simulink model "pgfm_ctrl_analysis"  (R2026b)
settings: Solver=ode23t  StopTime=param.sim.simlength  FixedStep=param.sim.tc  MaxStep=param.glb_time.tc  RelTol=1e-4
values from neighbouring files (symbols this model uses):
  param = add_template_extras(param, options)    [init_model.m]
undefined symbols (not defined in the file or in its folder): magnitude
libraries: fl_lib x99, nesl_utility x59, afe_uvw_ctrl x15, discrete_time_low_pass_filter x3, threephase_inductor_lib x3, dclink_for_two_levels x3, three_phase_pwm_modulator x3, ideal_bridges_lib x3, lithium_ion_battery x1, three_phase_voltage_with_frt_emulator_mfcn x1
(part 1 of 6)
settings Model: Creator=dbagn  LastModifiedBy=dbagn
settings SolverCC: SolverResetMethod=Robust  ZeroCrossControl=DisableAll
settings DataIOCC: DSMLogging=off  ReturnWorkspaceOutputs=off  SaveOutput=off  SaveTime=off  SignalLogging=off
settings OptimizationCC: ReuseModelBlockBuffer=off
settings SFSimCC: CustomCodeUndefinedFunction=ThrowError  DefaultCustomCodeDeterministicFunctions=All
settings SFSimCC: SimCustomHeaderCode=|
  | #include "rpi.h"
  | #include "rpi_simulink.h"
  | #include "bemf_obsv_load_est.h"
  | #include "bemf_obsv_load_est_simulink.h"
  | #include "dqpll_grid.h"
  | #include "dsmavgflt.h"
  | #include "bemf_obsv.h"
  | #include "bemf_obsv_simulink.h"
  | #include "mavgflt.h"
  | #include "mavgflt_simulink.h"
  | #include "mavgflts.h"
  | #include "mavgflts_simulink.h"
  | #include "sv_pwm_cm.h"
  | #include "dsmavgflt_simulink.h"
  | #include "linear_double_integrator_observer_simulink.h"
  | #include "sv_pwm_cm_simulink.h"
  | #include "dqvector_pi.h"
  | #include "dqpll_grid_simulink.h"
  | #include "first_harmonic_tracker.h"
  | #include "dqvector_pi_simulink.h"
  | #include "first_harmonic_tracker_simulink.h"
  | #include "dqpll_thyr.h"
  | #include "sv_pwm_simulink.h"
  | #include "sv_pwm.h"
  | #include "dqpll_thyr_simulink.h"
  | #include "linear_double_integrator_observer.h"
  | #include "math_f.h"
settings SFSimCC: SimUserIncludeDirs=|
  | include
  | src
settings SFSimCC: SimUserSources=|
  | "rpi.c"
  | "rpi_simulink.c"
  | "mavgflt_simulink.c"
  | "mavgflt.c"
  | "mavgflts_simulink.c"
  | "mavgflts.c"
  | "dsmavgflt_simulink.c"
  | "dsmavgflt.c"
  | "bemf_obsv_simulink.c"
  | "bemf_obsv.c"
  | "bemf_obsv_load_est_simulink.c"
  | "bemf_obsv_load_est.c"
  | "dqvector_pi.c"
  | "dqvector_pi_simulink.c"
  | "sv_pwm_simulink.c"
  | "sv_pwm.c"
  | "first_harmonic_tracker_simulink.c"
  | "first_harmonic_tracker.c"
  | "dqpll_thyr_simulink.c"
  | "dqpll_thyr.c"
  | "dqpll_grid_simulink.c"
  | "dqpll_grid.c"
  | "linear_double_integrator_observer_simulink.c"
  | "linear_double_integrator_observer.c"
  | "sv_pwm_cm_simulink.c"
  | "sv_pwm_cm.c"
settings RTWCC: DLArmComputeVersion=19.05
settings SimscapeCC: SimscapeUseEnergyAccounting=off

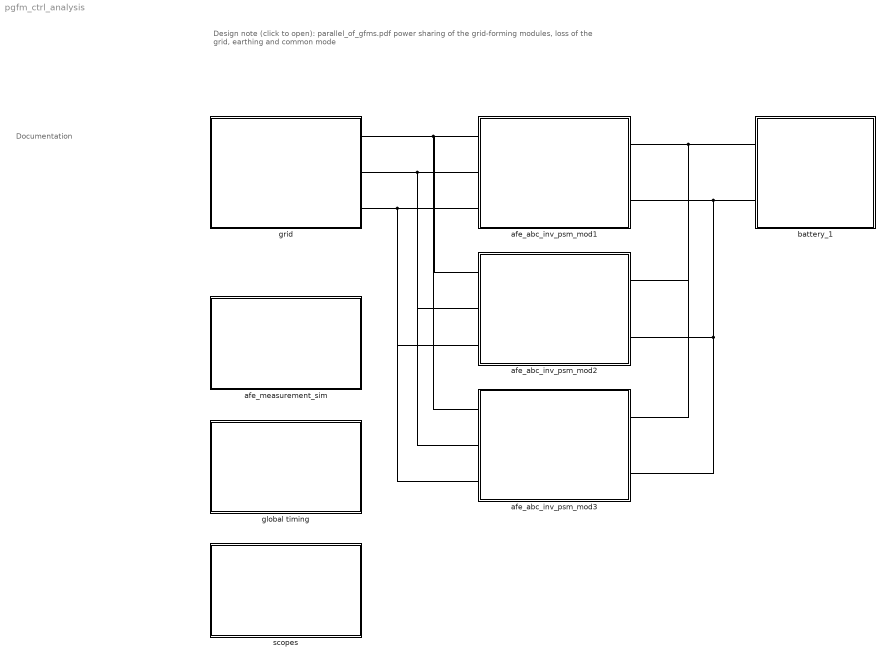
== system pgfm_ctrl_analysis ==
  note: Documentation
  note: Design note (click to open): parallel_of_gfms.pdf
      | power sharing of the grid-forming modules, loss of the grid, earthing and common mode
  afe_abc_inv_psm_mod1 : Subsystem
  afe_abc_inv_psm_mod2 : Subsystem
  afe_abc_inv_psm_mod3 : Subsystem
  afe_measurement_sim : Subsystem
  battery_1 : Subsystem
  global timing : Subsystem
  grid : Subsystem
  scopes : Subsystem
  connections:
  grid/RConn1 -- afe_abc_inv_psm_mod3/LConn1 -- afe_abc_inv_psm_mod2/LConn1 -- afe_abc_inv_psm_mod1/LConn1
  grid/RConn3 -- afe_abc_inv_psm_mod3/LConn3 -- afe_abc_inv_psm_mod2/LConn3 -- afe_abc_inv_psm_mod1/LConn3
  afe_abc_inv_psm_mod1/LConn2 -- afe_abc_inv_psm_mod3/LConn2 -- afe_abc_inv_psm_mod2/LConn2 -- grid/RConn2
  battery_1/RConn1 -- afe_abc_inv_psm_mod3/RConn1 -- afe_abc_inv_psm_mod2/RConn1 -- afe_abc_inv_psm_mod1/RConn1
  battery_1/RConn2 -- afe_abc_inv_psm_mod3/RConn2 -- afe_abc_inv_psm_mod2/RConn2 -- afe_abc_inv_psm_mod1/RConn2

== system pgfm_ctrl_analysis/afe_abc_inv_psm_mod1 ==
  AFE_control : Subsystem
  LCL_filter : Subsystem
  afe : Subsystem
  ug_a : PMIOPort  Side=Left
  ug_b : PMIOPort  Port=2  Side=Left
  ug_c : PMIOPort  Port=3  Side=Left
  Udc(+) : PMIOPort  Port=4  Side=Right
  Udc(-) : PMIOPort  Port=5  Side=Right
  wires:
  AFE_control/1(dabc_out) -> afe/1(dabc)
  connections:
  LCL_filter/LConn1 -- afe/LConn1
  LCL_filter/LConn2 -- afe/LConn2
  LCL_filter/LConn3 -- afe/LConn3
  ug_a/RConn1 -- LCL_filter/RConn1
  ug_b/RConn1 -- LCL_filter/RConn2
  ug_c/RConn1 -- LCL_filter/RConn3
  Udc(+)/RConn1 -- afe/RConn1
  afe/RConn2 -- Udc(-)/RConn1

== system pgfm_ctrl_analysis/afe_abc_inv_psm_mod2 ==
  AFE_control : Subsystem
  LCL_filter : Subsystem
  afe : Subsystem
  ug_a : PMIOPort  Side=Left
  ug_b : PMIOPort  Port=2  Side=Left
  ug_c : PMIOPort  Port=3  Side=Left
  Udc(+) : PMIOPort  Port=4  Side=Right
  Udc(-) : PMIOPort  Port=5  Side=Right
  wires:
  AFE_control/1(dabc_out) -> afe/1(dabc)
  connections:
  afe/RConn2 -- Udc(-)/RConn1
  Udc(+)/RConn1 -- afe/RConn1
  ug_c/RConn1 -- LCL_filter/RConn3
  ug_b/RConn1 -- LCL_filter/RConn2
  ug_a/RConn1 -- LCL_filter/RConn1
  LCL_filter/LConn3 -- afe/LConn3
  LCL_filter/LConn2 -- afe/LConn2
  LCL_filter/LConn1 -- afe/LConn1

== system pgfm_ctrl_analysis/afe_abc_inv_psm_mod3 ==
  AFE_control : Subsystem
  LCL_filter : Subsystem
  afe : Subsystem
  ug_a : PMIOPort  Side=Left
  ug_b : PMIOPort  Port=2  Side=Left
  ug_c : PMIOPort  Port=3  Side=Left
  Udc(+) : PMIOPort  Port=4  Side=Right
  Udc(-) : PMIOPort  Port=5  Side=Right
  wires:
  AFE_control/1(dabc_out) -> afe/1(dabc)
  connections:
  LCL_filter/LConn1 -- afe/LConn1
  LCL_filter/LConn2 -- afe/LConn2
  LCL_filter/LConn3 -- afe/LConn3
  ug_a/RConn1 -- LCL_filter/RConn1
  ug_b/RConn1 -- LCL_filter/RConn2
  ug_c/RConn1 -- LCL_filter/RConn3
  Udc(+)/RConn1 -- afe/RConn1
  afe/RConn2 -- Udc(-)/RConn1

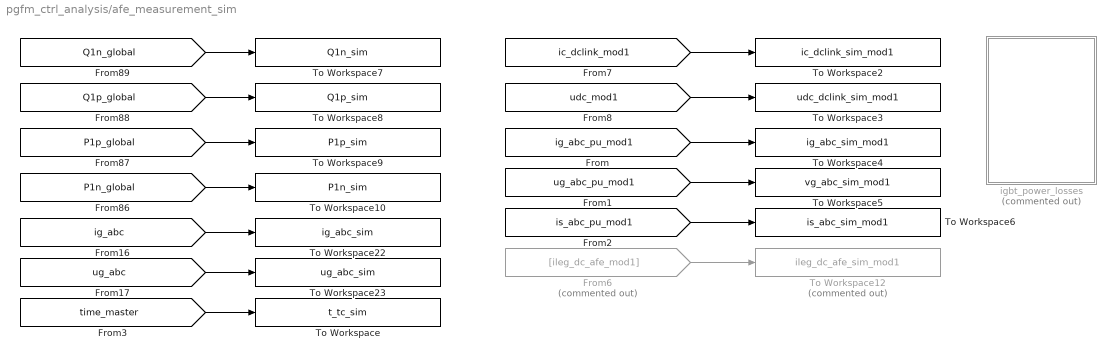
== system pgfm_ctrl_analysis/afe_measurement_sim ==
  From6 : From  Commented=on  GotoTag=ileg_dc_afe_mod1
  To Workspace : ToWorkspace  VariableName=t_tc_sim  SampleTime=param.glb_time.tc
      settings: MaxDataPoints=param.glb_time.Nc
  To Workspace10 : ToWorkspace  VariableName=P1n_sim  SampleTime=param.glb_time.ts_afe
      settings: MaxDataPoints=param.glb_time.Ns_afe
  To Workspace12 : ToWorkspace  Commented=on  VariableName=ileg_dc_afe_sim_mod1  SampleTime=param.glb_time.tc
      settings: MaxDataPoints=param.glb_time.Nc
  To Workspace2 : ToWorkspace  VariableName=ic_dclink_sim_mod1  SampleTime=param.glb_time.tc
      settings: MaxDataPoints=param.glb_time.Nc
  To Workspace22 : ToWorkspace  VariableName=ig_abc_sim  SampleTime=param.glb_time.tc
      settings: MaxDataPoints=param.glb_time.Nc
  To Workspace23 : ToWorkspace  VariableName=ug_abc_sim  SampleTime=param.glb_time.tc
      settings: MaxDataPoints=param.glb_time.Nc
  To Workspace3 : ToWorkspace  VariableName=udc_dclink_sim_mod1  SampleTime=param.glb_time.tc
      settings: MaxDataPoints=param.glb_time.Nc
  To Workspace4 : ToWorkspace  VariableName=ig_abc_sim_mod1  SampleTime=param.glb_time.tc
      settings: MaxDataPoints=param.glb_time.Nc
  To Workspace5 : ToWorkspace  VariableName=vg_abc_sim_mod1  SampleTime=param.glb_time.tc
      settings: MaxDataPoints=param.glb_time.Nc
  To Workspace6 : ToWorkspace  VariableName=is_abc_sim_mod1  SampleTime=param.glb_time.tc
      settings: MaxDataPoints=param.glb_time.Nc
  To Workspace7 : ToWorkspace  VariableName=Q1n_sim  SampleTime=param.glb_time.ts_afe
      settings: MaxDataPoints=param.glb_time.Ns_afe
  To Workspace8 : ToWorkspace  VariableName=Q1p_sim  SampleTime=param.glb_time.ts_afe
      settings: MaxDataPoints=param.glb_time.Ns_afe
  To Workspace9 : ToWorkspace  VariableName=P1p_sim  SampleTime=param.glb_time.ts_afe
      settings: MaxDataPoints=param.glb_time.Ns_afe
  igbt_power_losses : Subsystem  Commented=on
  wires:
  [time_master] -> To Workspace/1
  [Q1n_global] -> To Workspace7/1
  [Q1p_global] -> To Workspace8/1
  [P1p_global] -> To Workspace9/1
  [P1n_global] -> To Workspace10/1
  [ug_abc] -> To Workspace23/1
  [ig_abc] -> To Workspace22/1
  [ug_abc_pu_mod1] -> To Workspace5/1
  [ig_abc_pu_mod1] -> To Workspace4/1
  From6/1 -> To Workspace12/1
  [udc_mod1] -> To Workspace3/1
  [ic_dclink_mod1] -> To Workspace2/1
  [is_abc_pu_mod1] -> To Workspace6/1

== system pgfm_ctrl_analysis/battery_1 ==
  Electrical Reference1 : fl_lib/Electrical/Electrical Elements/Electrical Reference
  HF and Ground Network : Subsystem
  To Workspace14 : ToWorkspace  VariableName=battery_1_data_sim  SampleTime=param.glb_time.tc
      settings: MaxDataPoints=param.glb_time.Nc  Decimation=param.glb_time.decimation_tc
  lithium ion battery : Scope
      settings: ActiveDisplayYMinimum=-3613.5737689566768  ActiveDisplayYMaximum=22003.145712945909  DataLoggingVariableName=ScopeData3
  lithium_ion_battery : lithium_ion_battery/lithium_ion_battery  Q=param.battery.pack_1.Q  number_of_cells=param.battery.pack_1.number_of_cells  E_1=param.battery.pack_1.E_1  E0=param.battery.pack_1.E0  E1=param.battery.pack_1.E1  E2=param.battery.pack_1.E2  E3=param.battery.pack_1.E3  Elog=param.battery.pack_1.Elog  R0=param.battery.pack_1.R0  R1=param.battery.pack_1.R1  C1=param.battery.pack_1.C1  M=param.battery.pack_1.M  alpha=param.battery.pack_1.alpha  soc_init=param.battery.pack_1.soc_init  ts_battery=param.glb_time.ts_dab  q1Kalman=param.battery.pack_1.q1Kalman  q2Kalman=param.battery.pack_1.q2Kalman  q3Kalman=param.battery.pack_1.q3Kalman  rKalman=param.battery.pack_1.rKalman  tc=param.glb_time.tc  enable_white_noise_m=0  battery_voltage_init_m=param.battery.nominal_battery_voltage_1
  single_phase_ui_measure : Subsystem
  dc(+) : PMIOPort  Side=Right
  dc(-) : PMIOPort  Port=2  Side=Right
  wires:
  lithium_ion_battery/1 -> To Workspace14/1, lithium ion battery/1
  connections:
  single_phase_ui_measure/RConn1 -- dc(+)/RConn1
  single_phase_ui_measure/LConn1 -- HF and Ground Network/LConn1 -- lithium_ion_battery/RConn1
  dc(-)/RConn1 -- single_phase_ui_measure/RConn2
  single_phase_ui_measure/LConn2 -- HF and Ground Network/LConn2 -- lithium_ion_battery/RConn2
  HF and Ground Network/RConn1 -- Electrical Reference1/LConn1

== system pgfm_ctrl_analysis/global timing ==
  Unit Delay : UnitDelay  SampleTime=param.glb_time.tc
  Unit Delay1 : UnitDelay  SampleTime=param.glb_time.tc
  Unit Delay2 : UnitDelay  SampleTime=param.glb_time.tc
  time_afe1 : Subsystem  mask{k=param.afe.behav.time_gain_module_1}
      mask prompts: k "Time Gain"
      mask Display:
      | disp('time-gen');
      | port_label('input', 1, 'crt');
      | port_label('output', 1, 'tout');
  time_afe2 : Subsystem  mask{k=param.afe.behav.time_gain_module_2}
      mask prompts: k "Time Gain"
      mask Display:
      | disp('time-gen');
      | port_label('input', 1, 'crt');
      | port_label('output', 1, 'tout');
  time_afe3 : Subsystem  mask{k=param.afe.behav.time_gain_module_3}
      mask prompts: k "Time Gain"
      mask Display:
      | disp('time-gen');
      | port_label('input', 1, 'crt');
      | port_label('output', 1, 'tout');
  time_master : Subsystem  mask{k=1}
      mask prompts: k "Time Gain"
      mask Display:
      | disp('time-gen');
      | port_label('output', 1, 'tout');
  tag scope: time_afe_module_1=global, time_afe_module_2=global, time_afe_module_3=global, time_master=global
  wires:
  time_afe1/1(Out1) -> [time_afe_module_1]
  time_afe2/1(Out1) -> [time_afe_module_2]
  time_master/1(Out1) -> [time_master]
  [local_time_corr_afe1] -> Unit Delay/1
  Unit Delay/1 -> time_afe1/1(correction_time)
  [local_time_corr_afe2] -> Unit Delay1/1
  Unit Delay1/1 -> time_afe2/1(correction_time)
  [local_time_corr_afe3] -> Unit Delay2/1
  Unit Delay2/1 -> time_afe3/1(correction_time)
  time_afe3/1(Out1) -> [time_afe_module_3]

== system pgfm_ctrl_analysis/grid ==
  grid_emulator : Subsystem
  power meter iec mfunc : Subsystem
  threephase_vi_measures : Subsystem
  ua : PMIOPort  Side=Right
  ub : PMIOPort  Port=2  Side=Right
  uc : PMIOPort  Port=3  Side=Right
  connections:
  threephase_vi_measures/LConn3 -- grid_emulator/RConn3
  threephase_vi_measures/LConn1 -- grid_emulator/RConn1
  threephase_vi_measures/RConn2 -- ub/RConn1
  threephase_vi_measures/LConn2 -- grid_emulator/RConn2
  threephase_vi_measures/RConn1 -- ua/RConn1
  threephase_vi_measures/RConn3 -- uc/RConn1

== system pgfm_ctrl_analysis/scopes ==
  grid_afe_side : Subsystem
  igbt_power_losses : Subsystem  Commented=on
  mosfet_power_losses : Subsystem  Commented=on

== system pgfm_ctrl_analysis/afe_abc_inv_psm_mod1/AFE_control ==
  To Workspace : ToWorkspace  VariableName=afe_ctrl_data_output_mod1  SampleTime=param.glb_time.ts_afe
      settings: MaxDataPoints=param.glb_time.Ns_afe
  afe_control : Subsystem
  dabc_out : Outport
  tag scope: local_time_corr_afe1=global
  wires:
  [TRGO_afe_module_1] -> afe_control/Trigger
  [ug_abc_pu_mod1] -> afe_control/1(ug_abc_pu)
  [is_abc_pu_mod1] -> afe_control/4(is_abc_pu)
  [vdc_pu_afe_mod1] -> afe_control/2(udc_pu)
  afe_control/1(duvw) -> dabc_out/1
  [ig_abc_pu_mod1] -> afe_control/3(ig_abc_pu)
  [time_afe_module_1] -> afe_control/5(local_time)
  [time_master] -> afe_control/6(master_time)
  [phase_grid_emulator] -> afe_control/7(grid_phase)
  afe_control/3(m_data) -> To Workspace/1
  afe_control/2(AFE1_local_time_corr) -> [local_time_corr_afe1]

== system pgfm_ctrl_analysis/afe_abc_inv_psm_mod1/LCL_filter ==
  CFu1 : fl_lib/Electrical/Electrical Elements/Capacitor  c=param.afe.hw.CFu F  r=param.afe.hw.RCFu Ohm  g=0 1/Ohm  i_specify=off  i_priority=None  i=0 A  i_nominal_specify=off  i_nominal_value=1  i_nominal_unit=A  v_specify=off  v_priority=None  v=0 V  v_nominal_specify=off  v_nominal_value=1  v_nominal_unit=V  vc_specify=off  vc_priority=High  vc=0 V  vc_nominal_specify=off  vc_nominal_value=1  vc_nominal_unit=V
  CFu2 : fl_lib/Electrical/Electrical Elements/Capacitor  c=param.afe.hw.CFu F  r=param.afe.hw.RCFu Ohm  g=0 1/Ohm  i_specify=off  i_priority=None  i=0 A  i_nominal_specify=off  i_nominal_value=1  i_nominal_unit=A  v_specify=off  v_priority=None  v=0 V  v_nominal_specify=off  v_nominal_value=1  v_nominal_unit=V  vc_specify=off  vc_priority=High  vc=0 V  vc_nominal_specify=off  vc_nominal_value=1  vc_nominal_unit=V
  CFu3 : fl_lib/Electrical/Electrical Elements/Capacitor  c=param.afe.hw.CFu F  r=param.afe.hw.RCFu Ohm  g=0 1/Ohm  i_specify=off  i_priority=None  i=0 A  i_nominal_specify=off  i_nominal_value=1  i_nominal_unit=A  v_specify=off  v_priority=None  v=0 V  v_nominal_specify=off  v_nominal_value=1  v_nominal_unit=V  vc_specify=off  vc_priority=High  vc=0 V  vc_nominal_specify=off  vc_nominal_value=1  vc_nominal_unit=V
  Inductor : fl_lib/Electrical/Electrical Elements/Inductor  l=1e-6 H  r=0 Ohm  g=1e-9 1/Ohm  i_specify=on  i_priority=High  i=0 A  i_nominal_specify=off  i_nominal_value=1  i_nominal_unit=A  v_specify=off  v_priority=None  v=0 V  v_nominal_specify=off  v_nominal_value=1  v_nominal_unit=V  i_L_specify=off  i_L_priority=High  i_L=0 A  i_L_nominal_specify=off  i_L_nominal_value=1  i_L_nominal_unit=A
  Inductor1 : fl_lib/Electrical/Electrical Elements/Inductor  l=1e-6 H  r=0 Ohm  g=1e-9 1/Ohm  i_specify=on  i_priority=High  i=0 A  i_nominal_specify=off  i_nominal_value=1  i_nominal_unit=A  v_specify=off  v_priority=None  v=0 V  v_nominal_specify=off  v_nominal_value=1  v_nominal_unit=V  i_L_specify=off  i_L_priority=High  i_L=0 A  i_L_nominal_specify=off  i_L_nominal_value=1  i_L_nominal_unit=A
  Inductor2 : fl_lib/Electrical/Electrical Elements/Inductor  l=1e-6 H  r=0 Ohm  g=1e-9 1/Ohm  i_specify=on  i_priority=High  i=0 A  i_nominal_specify=off  i_nominal_value=1  i_nominal_unit=A  v_specify=off  v_priority=None  v=0 V  v_nominal_specify=off  v_nominal_value=1  v_nominal_unit=V  i_L_specify=off  i_L_priority=High  i_L=0 A  i_L_nominal_specify=off  i_L_nominal_value=1  i_L_nominal_unit=A
  threephase inductor : threephase_inductor_lib/threephase inductor  Lp=param.afe.hw.LFu H  L0=param.afe.hw.LFu_cm H  Rp=param.afe.hw.RLFu Ohm  R0=param.afe.hw.RLFu_cm Ohm  Lls=5e-6 H  uu_1_specify=off  uu_1_priority=None  uu_1=0 V  uu_1_nominal_specify=off  uu_1_nominal_value=1  uu_1_nominal_unit=V  uv_1_specify=off  uv_1_priority=None  uv_1=0 V  uv_1_nominal_specify=off  uv_1_nominal_value=1  uv_1_nominal_unit=V  uw_1_specify=off  uw_1_priority=None  uw_1=0 V  uw_1_nominal_specify=off  uw_1_nominal_value=1  uw_1_nominal_unit=V  uu_2_specify=off  uu_2_priority=None  uu_2=0 V  uu_2_nominal_specify=off  uu_2_nominal_value=1  uu_2_nominal_unit=V  uv_2_specify=off  uv_2_priority=None  uv_2=0 V  uv_2_nominal_specify=off  uv_2_nominal_value=1  uv_2_nominal_unit=V  uw_2_specify=off  uw_2_priority=None  uw_2=0 V  uw_2_nominal_specify=off  uw_2_nominal_value=1  uw_2_nominal_unit=V  iu_specify=off  iu_priority=High  iu=0 A  iu_nominal_specify=off  iu_nominal_value=1  iu_nominal_unit=A  iv_specify=off  iv_priority=High  iv=0 A  iv_nominal_specify=off  iv_nominal_value=1  iv_nominal_unit=A  iw_specify=off  iw_priority=High  iw=0 A  iw_nominal_specify=off  iw_nominal_value=1  iw_nominal_unit=A
  threephase_vi_measures_stack : Subsystem
  threephase_vi_measures_stack1 : Subsystem
  us_a : PMIOPort  Side=Left
  ug_a : PMIOPort  Port=2  Side=Right
  us_b : PMIOPort  Port=3  Side=Left
  ug_b : PMIOPort  Port=4  Side=Right
  us_c : PMIOPort  Port=5  Side=Left
  ug_c : PMIOPort  Port=6  Side=Right
  connections:
  CFu1/RConn1 -- CFu3/RConn1 -- CFu2/RConn1
  Inductor/RConn1 -- threephase_vi_measures_stack1/LConn1 -- CFu1/LConn1
  Inductor2/RConn1 -- CFu3/LConn1 -- threephase_vi_measures_stack1/LConn3
  Inductor1/RConn1 -- CFu2/LConn1 -- threephase_vi_measures_stack1/LConn2
  threephase_vi_measures_stack/LConn1 -- us_a/RConn1
  threephase_vi_measures_stack/LConn2 -- us_b/RConn1
  threephase_vi_measures_stack/LConn3 -- us_c/RConn1
  threephase_vi_measures_stack/RConn1 -- threephase inductor/LConn1
  threephase_vi_measures_stack/RConn2 -- threephase inductor/LConn2
  threephase_vi_measures_stack/RConn3 -- threephase inductor/LConn3
  threephase inductor/RConn1 -- Inductor/LConn1
  Inductor1/LConn1 -- threephase inductor/RConn2
  Inductor2/LConn1 -- threephase inductor/RConn3
  ug_a/RConn1 -- threephase_vi_measures_stack1/RConn1
  ug_b/RConn1 -- threephase_vi_measures_stack1/RConn2
  ug_c/RConn1 -- threephase_vi_measures_stack1/RConn3

== system pgfm_ctrl_analysis/afe_abc_inv_psm_mod1/afe ==
  dabc : Inport
  Bus Selector : BusSelector  OutputSignals=vdc_pu
  Bus Selector1 : BusSelector  OutputSignals=udc,udc_p_gnd,udc_centertap_gnd,udc_n_gnd  OutputAsBus=on
  Bus Selector2 : BusSelector  OutputSignals=udc
  Bus Selector3 : BusSelector  OutputSignals=Cdc1_current
  dclink1 : dclink_for_two_levels/dclink  Cdc=param.afe.hw.CFi  Rudc_measure=1e6  Vdc_scale=param.afe.hw.udc_nom
  sv_pwm : Subsystem
  three_phase_inverter_ideal_switch_based_model : Subsystem
  us_a : PMIOPort  Side=Left
  us_b : PMIOPort  Port=2  Side=Left
  us_c : PMIOPort  Port=3  Side=Left
  Udc(+) : PMIOPort  Port=4  Side=Right
  Udc(-) : PMIOPort  Port=5  Side=Right
  tag scope: all_voltages_about_dclink=global, ic_dclink_mod1=global, udc_mod1=global, vdc_pu_afe_mod1=global, vdc_pu_inv_mod1=global
  wires:
  dabc/1 -> sv_pwm/1(duties_uvw)
  sv_pwm/1(gate_cmds) -> three_phase_inverter_ideal_switch_based_model/1(gate_commands)
  dclink1/1 -> Bus Selector1/1, Bus Selector2/1, Bus Selector3/1, Bus Selector/1
  Bus Selector1/1 -> [all_voltages_about_dclink]
  Bus Selector/1 -> [vdc_pu_afe_mod1], [vdc_pu_inv_mod1]  "<vdc_pu>"
  Bus Selector2/1 -> [udc_mod1]  "<udc>"
  Bus Selector3/1 -> [ic_dclink_mod1]  "<Cdc1_current>"
  connections:
  three_phase_inverter_ideal_switch_based_model/RConn2 -- us_b/RConn1
  dclink1/RConn1 -- Udc(+)/RConn1
  dclink1/RConn2 -- Udc(-)/RConn1
  three_phase_inverter_ideal_switch_based_model/RConn1 -- us_a/RConn1
  three_phase_inverter_ideal_switch_based_model/RConn3 -- us_c/RConn1
  dclink1/LConn2 -- three_phase_inverter_ideal_switch_based_model/LConn2
  dclink1/LConn1 -- three_phase_inverter_ideal_switch_based_model/LConn1

== system pgfm_ctrl_analysis/afe_abc_inv_psm_mod2/AFE_control ==
  To Workspace : ToWorkspace  VariableName=afe_ctrl_data_output_mod2  SampleTime=param.glb_time.ts_afe
      settings: MaxDataPoints=param.glb_time.Ns_afe
  afe_control : Subsystem
  dabc_out : Outport
  tag scope: local_time_corr_afe2=global
  wires:
  afe_control/2(AFE1_local_time_corr) -> [local_time_corr_afe2]
  afe_control/3(m_data) -> To Workspace/1
  [phase_grid_emulator] -> afe_control/7(grid_phase)
  [time_master] -> afe_control/6(master_time)
  [time_afe_module_2] -> afe_control/5(local_time)
  [ig_abc_pu_mod2] -> afe_control/3(ig_abc_pu)
  afe_control/1(duvw) -> dabc_out/1
  [vdc_pu_afe_mod2] -> afe_control/2(udc_pu)
  [is_abc_pu_mod2] -> afe_control/4(is_abc_pu)
  [ug_abc_pu_mod2] -> afe_control/1(ug_abc_pu)
  [TRGO_afe_module_2] -> afe_control/Trigger

== system pgfm_ctrl_analysis/afe_abc_inv_psm_mod2/LCL_filter ==
  CFu1 : fl_lib/Electrical/Electrical Elements/Capacitor  c=param.afe.hw.CFu F  r=param.afe.hw.RCFu Ohm  g=0 1/Ohm  i_specify=off  i_priority=None  i=0 A  i_nominal_specify=off  i_nominal_value=1  i_nominal_unit=A  v_specify=off  v_priority=None  v=0 V  v_nominal_specify=off  v_nominal_value=1  v_nominal_unit=V  vc_specify=off  vc_priority=High  vc=0 V  vc_nominal_specify=off  vc_nominal_value=1  vc_nominal_unit=V
  CFu2 : fl_lib/Electrical/Electrical Elements/Capacitor  c=param.afe.hw.CFu F  r=param.afe.hw.RCFu Ohm  g=0 1/Ohm  i_specify=off  i_priority=None  i=0 A  i_nominal_specify=off  i_nominal_value=1  i_nominal_unit=A  v_specify=off  v_priority=None  v=0 V  v_nominal_specify=off  v_nominal_value=1  v_nominal_unit=V  vc_specify=off  vc_priority=High  vc=0 V  vc_nominal_specify=off  vc_nominal_value=1  vc_nominal_unit=V
  CFu3 : fl_lib/Electrical/Electrical Elements/Capacitor  c=param.afe.hw.CFu F  r=param.afe.hw.RCFu Ohm  g=0 1/Ohm  i_specify=off  i_priority=None  i=0 A  i_nominal_specify=off  i_nominal_value=1  i_nominal_unit=A  v_specify=off  v_priority=None  v=0 V  v_nominal_specify=off  v_nominal_value=1  v_nominal_unit=V  vc_specify=off  vc_priority=High  vc=0 V  vc_nominal_specify=off  vc_nominal_value=1  vc_nominal_unit=V
  Inductor : fl_lib/Electrical/Electrical Elements/Inductor  l=1e-6 H  r=0 Ohm  g=1e-9 1/Ohm  i_specify=on  i_priority=High  i=0 A  i_nominal_specify=off  i_nominal_value=1  i_nominal_unit=A  v_specify=off  v_priority=None  v=0 V  v_nominal_specify=off  v_nominal_value=1  v_nominal_unit=V  i_L_specify=off  i_L_priority=High  i_L=0 A  i_L_nominal_specify=off  i_L_nominal_value=1  i_L_nominal_unit=A
  Inductor1 : fl_lib/Electrical/Electrical Elements/Inductor  l=1e-6 H  r=0 Ohm  g=1e-9 1/Ohm  i_specify=on  i_priority=High  i=0 A  i_nominal_specify=off  i_nominal_value=1  i_nominal_unit=A  v_specify=off  v_priority=None  v=0 V  v_nominal_specify=off  v_nominal_value=1  v_nominal_unit=V  i_L_specify=off  i_L_priority=High  i_L=0 A  i_L_nominal_specify=off  i_L_nominal_value=1  i_L_nominal_unit=A
  Inductor2 : fl_lib/Electrical/Electrical Elements/Inductor  l=1e-6 H  r=0 Ohm  g=1e-9 1/Ohm  i_specify=on  i_priority=High  i=0 A  i_nominal_specify=off  i_nominal_value=1  i_nominal_unit=A  v_specify=off  v_priority=None  v=0 V  v_nominal_specify=off  v_nominal_value=1  v_nominal_unit=V  i_L_specify=off  i_L_priority=High  i_L=0 A  i_L_nominal_specify=off  i_L_nominal_value=1  i_L_nominal_unit=A
  threephase inductor : threephase_inductor_lib/threephase inductor  Lp=param.afe.hw.LFu H  L0=param.afe.hw.LFu_cm H  Rp=param.afe.hw.RLFu Ohm  R0=param.afe.hw.RLFu_cm Ohm  Lls=5e-6 H  uu_1_specify=off  uu_1_priority=None  uu_1=0 V  uu_1_nominal_specify=off  uu_1_nominal_value=1  uu_1_nominal_unit=V  uv_1_specify=off  uv_1_priority=None  uv_1=0 V  uv_1_nominal_specify=off  uv_1_nominal_value=1  uv_1_nominal_unit=V  uw_1_specify=off  uw_1_priority=None  uw_1=0 V  uw_1_nominal_specify=off  uw_1_nominal_value=1  uw_1_nominal_unit=V  uu_2_specify=off  uu_2_priority=None  uu_2=0 V  uu_2_nominal_specify=off  uu_2_nominal_value=1  uu_2_nominal_unit=V  uv_2_specify=off  uv_2_priority=None  uv_2=0 V  uv_2_nominal_specify=off  uv_2_nominal_value=1  uv_2_nominal_unit=V  uw_2_specify=off  uw_2_priority=None  uw_2=0 V  uw_2_nominal_specify=off  uw_2_nominal_value=1  uw_2_nominal_unit=V  iu_specify=off  iu_priority=High  iu=0 A  iu_nominal_specify=off  iu_nominal_value=1  iu_nominal_unit=A  iv_specify=off  iv_priority=High  iv=0 A  iv_nominal_specify=off  iv_nominal_value=1  iv_nominal_unit=A  iw_specify=off  iw_priority=High  iw=0 A  iw_nominal_specify=off  iw_nominal_value=1  iw_nominal_unit=A
  threephase_vi_measures_stack : Subsystem
  threephase_vi_measures_stack1 : Subsystem
  us_a : PMIOPort  Side=Left
  ug_a : PMIOPort  Port=2  Side=Right
  us_b : PMIOPort  Port=3  Side=Left
  ug_b : PMIOPort  Port=4  Side=Right
  us_c : PMIOPort  Port=5  Side=Left
  ug_c : PMIOPort  Port=6  Side=Right
  connections:
  ug_c/RConn1 -- threephase_vi_measures_stack1/RConn3
  ug_b/RConn1 -- threephase_vi_measures_stack1/RConn2
  ug_a/RConn1 -- threephase_vi_measures_stack1/RConn1
  Inductor2/LConn1 -- threephase inductor/RConn3
  Inductor1/LConn1 -- threephase inductor/RConn2
  threephase inductor/RConn1 -- Inductor/LConn1
  threephase_vi_measures_stack/RConn3 -- threephase inductor/LConn3
  threephase_vi_measures_stack/RConn2 -- threephase inductor/LConn2
  threephase_vi_measures_stack/RConn1 -- threephase inductor/LConn1
  threephase_vi_measures_stack/LConn3 -- us_c/RConn1
  threephase_vi_measures_stack/LConn2 -- us_b/RConn1
  threephase_vi_measures_stack/LConn1 -- us_a/RConn1
  threephase_vi_measures_stack1/LConn2 -- CFu2/LConn1 -- Inductor1/RConn1
  threephase_vi_measures_stack1/LConn3 -- CFu3/LConn1 -- Inductor2/RConn1
  CFu1/LConn1 -- threephase_vi_measures_stack1/LConn1 -- Inductor/RConn1
  CFu2/RConn1 -- CFu3/RConn1 -- CFu1/RConn1

== system pgfm_ctrl_analysis/afe_abc_inv_psm_mod2/afe ==
  dabc : Inport
  Bus Selector : BusSelector  OutputSignals=vdc_pu
  Bus Selector1 : BusSelector  OutputSignals=udc,udc_p_gnd,udc_centertap_gnd,udc_n_gnd  OutputAsBus=on
  Bus Selector2 : BusSelector  OutputSignals=udc
  Bus Selector3 : BusSelector  OutputSignals=Cdc1_current
  dclink1 : dclink_for_two_levels/dclink  Cdc=param.afe.hw.CFi  Rudc_measure=1e6  Vdc_scale=param.afe.hw.udc_nom
  sv_pwm : Subsystem
  three_phase_inverter_ideal_switch_based_model : Subsystem
  us_a : PMIOPort  Side=Left
  us_b : PMIOPort  Port=2  Side=Left
  us_c : PMIOPort  Port=3  Side=Left
  Udc(+) : PMIOPort  Port=4  Side=Right
  Udc(-) : PMIOPort  Port=5  Side=Right
  tag scope: all_voltages_about_dclink_mod2=global, ic_dclink_mod2=global, udc_mod2=global, vdc_pu_afe_mod2=global, vdc_pu_inv_mod2=global
  wires:
  Bus Selector3/1 -> [ic_dclink_mod2]  "<Cdc1_current>"
  Bus Selector2/1 -> [udc_mod2]  "<udc>"
  Bus Selector/1 -> [vdc_pu_inv_mod2], [vdc_pu_afe_mod2]  "<vdc_pu>"
  Bus Selector1/1 -> [all_voltages_about_dclink_mod2]
  dclink1/1 -> Bus Selector/1, Bus Selector3/1, Bus Selector2/1, Bus Selector1/1
  sv_pwm/1(gate_cmds) -> three_phase_inverter_ideal_switch_based_model/1(gate_commands)
  dabc/1 -> sv_pwm/1(duties_uvw)
  connections:
  dclink1/LConn1 -- three_phase_inverter_ideal_switch_based_model/LConn1
  dclink1/LConn2 -- three_phase_inverter_ideal_switch_based_model/LConn2
  three_phase_inverter_ideal_switch_based_model/RConn3 -- us_c/RConn1
  three_phase_inverter_ideal_switch_based_model/RConn1 -- us_a/RConn1
  dclink1/RConn2 -- Udc(-)/RConn1
  dclink1/RConn1 -- Udc(+)/RConn1
  three_phase_inverter_ideal_switch_based_model/RConn2 -- us_b/RConn1

== system pgfm_ctrl_analysis/afe_abc_inv_psm_mod3/AFE_control ==
  To Workspace : ToWorkspace  VariableName=afe_ctrl_data_output_mod3  SampleTime=param.glb_time.ts_afe
      settings: MaxDataPoints=param.glb_time.Ns_afe
  afe_control : Subsystem
  dabc_out : Outport
  tag scope: local_time_corr_afe3=global
  wires:
  [TRGO_afe_module_3] -> afe_control/Trigger
  [ug_abc_pu_mod3] -> afe_control/1(ug_abc_pu)
  [is_abc_pu_mod3] -> afe_control/4(is_abc_pu)
  [vdc_pu_afe_mod3] -> afe_control/2(udc_pu)
  afe_control/1(duvw) -> dabc_out/1
  [ig_abc_pu_mod3] -> afe_control/3(ig_abc_pu)
  [time_afe_module_3] -> afe_control/5(local_time)
  [time_master] -> afe_control/6(master_time)
  [phase_grid_emulator] -> afe_control/7(grid_phase)
  afe_control/3(m_data) -> To Workspace/1
  afe_control/2(AFE1_local_time_corr) -> [local_time_corr_afe3]

== system pgfm_ctrl_analysis/afe_abc_inv_psm_mod3/LCL_filter ==
  CFu1 : fl_lib/Electrical/Electrical Elements/Capacitor  c=param.afe.hw.CFu F  r=param.afe.hw.RCFu Ohm  g=0 1/Ohm  i_specify=off  i_priority=None  i=0 A  i_nominal_specify=off  i_nominal_value=1  i_nominal_unit=A  v_specify=off  v_priority=None  v=0 V  v_nominal_specify=off  v_nominal_value=1  v_nominal_unit=V  vc_specify=off  vc_priority=High  vc=0 V  vc_nominal_specify=off  vc_nominal_value=1  vc_nominal_unit=V
  CFu2 : fl_lib/Electrical/Electrical Elements/Capacitor  c=param.afe.hw.CFu F  r=param.afe.hw.RCFu Ohm  g=0 1/Ohm  i_specify=off  i_priority=None  i=0 A  i_nominal_specify=off  i_nominal_value=1  i_nominal_unit=A  v_specify=off  v_priority=None  v=0 V  v_nominal_specify=off  v_nominal_value=1  v_nominal_unit=V  vc_specify=off  vc_priority=High  vc=0 V  vc_nominal_specify=off  vc_nominal_value=1  vc_nominal_unit=V
  CFu3 : fl_lib/Electrical/Electrical Elements/Capacitor  c=param.afe.hw.CFu F  r=param.afe.hw.RCFu Ohm  g=0 1/Ohm  i_specify=off  i_priority=None  i=0 A  i_nominal_specify=off  i_nominal_value=1  i_nominal_unit=A  v_specify=off  v_priority=None  v=0 V  v_nominal_specify=off  v_nominal_value=1  v_nominal_unit=V  vc_specify=off  vc_priority=High  vc=0 V  vc_nominal_specify=off  vc_nominal_value=1  vc_nominal_unit=V
  Inductor : fl_lib/Electrical/Electrical Elements/Inductor  l=1e-6 H  r=0 Ohm  g=1e-9 1/Ohm  i_specify=on  i_priority=High  i=0 A  i_nominal_specify=off  i_nominal_value=1  i_nominal_unit=A  v_specify=off  v_priority=None  v=0 V  v_nominal_specify=off  v_nominal_value=1  v_nominal_unit=V  i_L_specify=off  i_L_priority=High  i_L=0 A  i_L_nominal_specify=off  i_L_nominal_value=1  i_L_nominal_unit=A
  Inductor1 : fl_lib/Electrical/Electrical Elements/Inductor  l=1e-6 H  r=0 Ohm  g=1e-9 1/Ohm  i_specify=on  i_priority=High  i=0 A  i_nominal_specify=off  i_nominal_value=1  i_nominal_unit=A  v_specify=off  v_priority=None  v=0 V  v_nominal_specify=off  v_nominal_value=1  v_nominal_unit=V  i_L_specify=off  i_L_priority=High  i_L=0 A  i_L_nominal_specify=off  i_L_nominal_value=1  i_L_nominal_unit=A
  Inductor2 : fl_lib/Electrical/Electrical Elements/Inductor  l=1e-6 H  r=0 Ohm  g=1e-9 1/Ohm  i_specify=on  i_priority=High  i=0 A  i_nominal_specify=off  i_nominal_value=1  i_nominal_unit=A  v_specify=off  v_priority=None  v=0 V  v_nominal_specify=off  v_nominal_value=1  v_nominal_unit=V  i_L_specify=off  i_L_priority=High  i_L=0 A  i_L_nominal_specify=off  i_L_nominal_value=1  i_L_nominal_unit=A
  threephase inductor : threephase_inductor_lib/threephase inductor  Lp=param.afe.hw.LFu H  L0=param.afe.hw.LFu_cm H  Rp=param.afe.hw.RLFu Ohm  R0=param.afe.hw.RLFu_cm Ohm  Lls=5e-6 H  uu_1_specify=off  uu_1_priority=None  uu_1=0 V  uu_1_nominal_specify=off  uu_1_nominal_value=1  uu_1_nominal_unit=V  uv_1_specify=off  uv_1_priority=None  uv_1=0 V  uv_1_nominal_specify=off  uv_1_nominal_value=1  uv_1_nominal_unit=V  uw_1_specify=off  uw_1_priority=None  uw_1=0 V  uw_1_nominal_specify=off  uw_1_nominal_value=1  uw_1_nominal_unit=V  uu_2_specify=off  uu_2_priority=None  uu_2=0 V  uu_2_nominal_specify=off  uu_2_nominal_value=1  uu_2_nominal_unit=V  uv_2_specify=off  uv_2_priority=None  uv_2=0 V  uv_2_nominal_specify=off  uv_2_nominal_value=1  uv_2_nominal_unit=V  uw_2_specify=off  uw_2_priority=None  uw_2=0 V  uw_2_nominal_specify=off  uw_2_nominal_value=1  uw_2_nominal_unit=V  iu_specify=off  iu_priority=High  iu=0 A  iu_nominal_specify=off  iu_nominal_value=1  iu_nominal_unit=A  iv_specify=off  iv_priority=High  iv=0 A  iv_nominal_specify=off  iv_nominal_value=1  iv_nominal_unit=A  iw_specify=off  iw_priority=High  iw=0 A  iw_nominal_specify=off  iw_nominal_value=1  iw_nominal_unit=A
  threephase_vi_measures_stack : Subsystem
  threephase_vi_measures_stack1 : Subsystem
  us_a : PMIOPort  Side=Left
  ug_a : PMIOPort  Port=2  Side=Right
  us_b : PMIOPort  Port=3  Side=Left
  ug_b : PMIOPort  Port=4  Side=Right
  us_c : PMIOPort  Port=5  Side=Left
  ug_c : PMIOPort  Port=6  Side=Right
  connections:
  CFu1/RConn1 -- CFu3/RConn1 -- CFu2/RConn1
  Inductor/RConn1 -- threephase_vi_measures_stack1/LConn1 -- CFu1/LConn1
  Inductor2/RConn1 -- CFu3/LConn1 -- threephase_vi_measures_stack1/LConn3
  Inductor1/RConn1 -- CFu2/LConn1 -- threephase_vi_measures_stack1/LConn2
  threephase_vi_measures_stack/LConn1 -- us_a/RConn1
  threephase_vi_measures_stack/LConn2 -- us_b/RConn1
  threephase_vi_measures_stack/LConn3 -- us_c/RConn1
  threephase_vi_measures_stack/RConn1 -- threephase inductor/LConn1
  threephase_vi_measures_stack/RConn2 -- threephase inductor/LConn2
  threephase_vi_measures_stack/RConn3 -- threephase inductor/LConn3
  threephase inductor/RConn1 -- Inductor/LConn1
  Inductor1/LConn1 -- threephase inductor/RConn2
  Inductor2/LConn1 -- threephase inductor/RConn3
  ug_a/RConn1 -- threephase_vi_measures_stack1/RConn1
  ug_b/RConn1 -- threephase_vi_measures_stack1/RConn2
  ug_c/RConn1 -- threephase_vi_measures_stack1/RConn3

== system pgfm_ctrl_analysis/afe_abc_inv_psm_mod3/afe ==
  dabc : Inport
  Bus Selector : BusSelector  OutputSignals=vdc_pu
  Bus Selector1 : BusSelector  OutputSignals=udc,udc_p_gnd,udc_centertap_gnd,udc_n_gnd  OutputAsBus=on
  Bus Selector2 : BusSelector  OutputSignals=udc
  Bus Selector3 : BusSelector  OutputSignals=Cdc1_current
  dclink1 : dclink_for_two_levels/dclink  Cdc=param.afe.hw.CFi  Rudc_measure=1e6  Vdc_scale=param.afe.hw.udc_nom
  sv_pwm : Subsystem
  three_phase_inverter_ideal_switch_based_model : Subsystem
  us_a : PMIOPort  Side=Left
  us_b : PMIOPort  Port=2  Side=Left
  us_c : PMIOPort  Port=3  Side=Left
  Udc(+) : PMIOPort  Port=4  Side=Right
  Udc(-) : PMIOPort  Port=5  Side=Right
  tag scope: all_voltages_about_dclink_mod3=global, ic_dclink_mod3=global, udc_mod3=global, vdc_pu_afe_mod3=global, vdc_pu_inv_mod3=global
  wires:
  dabc/1 -> sv_pwm/1(duties_uvw)
  sv_pwm/1(gate_cmds) -> three_phase_inverter_ideal_switch_based_model/1(gate_commands)
  dclink1/1 -> Bus Selector1/1, Bus Selector2/1, Bus Selector3/1, Bus Selector/1
  Bus Selector1/1 -> [all_voltages_about_dclink_mod3]
  Bus Selector/1 -> [vdc_pu_afe_mod3], [vdc_pu_inv_mod3]  "<vdc_pu>"
  Bus Selector2/1 -> [udc_mod3]  "<udc>"
  Bus Selector3/1 -> [ic_dclink_mod3]  "<Cdc1_current>"
  connections:
  three_phase_inverter_ideal_switch_based_model/RConn2 -- us_b/RConn1
  dclink1/RConn1 -- Udc(+)/RConn1
  dclink1/RConn2 -- Udc(-)/RConn1
  three_phase_inverter_ideal_switch_based_model/RConn1 -- us_a/RConn1
  three_phase_inverter_ideal_switch_based_model/RConn3 -- us_c/RConn1
  dclink1/LConn2 -- three_phase_inverter_ideal_switch_based_model/LConn2
  dclink1/LConn1 -- three_phase_inverter_ideal_switch_based_model/LConn1

== system pgfm_ctrl_analysis/afe_measurement_sim/igbt_power_losses ==
  To Workspace1 : ToWorkspace  VariableName=igbt_ploss_afeQ1_sim  SampleTime=param.glb_time.tc
      settings: MaxDataPoints=param.glb_time.Nc
  To Workspace14 : ToWorkspace  VariableName=igbt_current_afeQ1_sim  SampleTime=param.glb_time.tc
      settings: MaxDataPoints=param.glb_time.Nc
  To Workspace15 : ToWorkspace  VariableName=igbt_voltage_afeQ1_sim  SampleTime=param.glb_time.tc
      settings: MaxDataPoints=param.glb_time.Nc
  To Workspace16 : ToWorkspace  VariableName=igbt_JH_temp_afeQ1_sim  SampleTime=param.glb_time.tc
      settings: MaxDataPoints=param.glb_time.Nc
  To Workspace17 : ToWorkspace  VariableName=igbt_HA_temp_afeQ1_sim  SampleTime=param.glb_time.tc
      settings: MaxDataPoints=param.glb_time.Nc
  To Workspace18 : ToWorkspace  VariableName=diode_ploss_afeQ1_sim  SampleTime=param.glb_time.tc
      settings: MaxDataPoints=param.glb_time.Nc
  To Workspace19 : ToWorkspace  VariableName=diode_JH_temp_afeQ1_sim  SampleTime=param.glb_time.tc
      settings: MaxDataPoints=param.glb_time.Nc
  To Workspace20 : ToWorkspace  VariableName=diode_HA_temp_afeQ1_sim  SampleTime=param.glb_time.tc
      settings: MaxDataPoints=param.glb_time.Nc
  wires:
  [igbt_JH_temp_afeQ1] -> To Workspace16/1  "igbt_JH_temp_afeQ1"
  [igbt_ploss_afeQ1] -> To Workspace1/1  "igbt_ploss_afeQ1"
  [igbt_HA_temp_afeQ1] -> To Workspace17/1  "igbt_HA_temp_afeQ1"
  [diode_ploss_afeQ1] -> To Workspace18/1  "diode_ploss_afeQ1"
  [igbt_current_afeQ1] -> To Workspace14/1  "igbt_current_afeQ1"
  [diode_JH_temp_afeQ1] -> To Workspace19/1  "diode_JH_temp_afeQ1"
  [igbt_voltage_afeQ1] -> To Workspace15/1  "igbt_voltage_afeQ1"
  [diode_JH_temp_afeQ1] -> To Workspace20/1  "diode_HA_temp_afeQ1"

== system pgfm_ctrl_analysis/battery_1/HF and Ground Network ==
  Capacitor : fl_lib/Electrical/Electrical Elements/Capacitor  c=param.gnd.c_batt_pole F  r=param.gnd.r_batt_hf Ohm  g=0 1/Ohm  i_specify=off  i_priority=None  i=0 A  i_nominal_specify=off  i_nominal_value=1  i_nominal_unit=A  v_specify=off  v_priority=None  v=0 V  v_nominal_specify=off  v_nominal_value=1  v_nominal_unit=V  vc_specify=off  vc_priority=High  vc=0 V  vc_nominal_specify=off  vc_nominal_value=1  vc_nominal_unit=V
  Capacitor1 : fl_lib/Electrical/Electrical Elements/Capacitor  c=param.gnd.c_batt_pole F  r=param.gnd.r_batt_hf Ohm  g=0 1/Ohm  i_specify=off  i_priority=None  i=0 A  i_nominal_specify=off  i_nominal_value=1  i_nominal_unit=A  v_specify=off  v_priority=None  v=0 V  v_nominal_specify=off  v_nominal_value=1  v_nominal_unit=V  vc_specify=off  vc_priority=High  vc=0 V  vc_nominal_specify=off  vc_nominal_value=1  vc_nominal_unit=V
  PS-Simulink Converter : nesl_utility/PS-Simulink Converter  PhysicalDomain=network_engine_domain  SubClassName=ps_output  LeftPortType=input  RightPortType=output  PseudoPeriodic=off  Frequencies=[]  VectorFormat=1-D array  Unit=V  AffineConversion=off
  PS-Simulink Converter1 : nesl_utility/PS-Simulink Converter  PhysicalDomain=network_engine_domain  SubClassName=ps_output  LeftPortType=input  RightPortType=output  PseudoPeriodic=off  Frequencies=[]  VectorFormat=1-D array  Unit=V  AffineConversion=off
  Resistor2 : fl_lib/Electrical/Electrical Elements/Resistor  R=param.gnd.r_gnd_pole Ohm  i_specify=off  i_priority=None  i=0 A  i_nominal_specify=off  i_nominal_value=1  i_nominal_unit=A  v_specify=off  v_priority=None  v=0 V  v_nominal_specify=off  v_nominal_value=1  v_nominal_unit=V
  Resistor3 : fl_lib/Electrical/Electrical Elements/Resistor  R=param.gnd.r_gnd_pole Ohm  i_specify=off  i_priority=None  i=0 A  i_nominal_specify=off  i_nominal_value=1  i_nominal_unit=A  v_specify=off  v_priority=None  v=0 V  v_nominal_specify=off  v_nominal_value=1  v_nominal_unit=V
  Time Scope : Scope  NumInputPorts=2
      settings: TimeUnits=Metric (based on Time Span)  ActiveDisplayYMinimum=-1656.2258944810565  ActiveDisplayYMaximum=1581.1518985778969  YLabel=Amplitude  DataLoggingVariableName=ScopeData4
  Voltage Sensor : fl_lib/Electrical/Electrical Sensors/Voltage Sensor
  Voltage Sensor1 : fl_lib/Electrical/Electrical Sensors/Voltage Sensor
  Udc(+) : PMIOPort  Side=Left
  Udc(-) : PMIOPort  Port=2  Side=Left
  gnd : PMIOPort  Port=3  Side=Right
  wires:
  PS-Simulink Converter/1 -> Time Scope/1
  PS-Simulink Converter1/1 -> Time Scope/2
  connections:
  Voltage Sensor1/RConn1 -- PS-Simulink Converter1/LConn1
  Voltage Sensor/RConn1 -- PS-Simulink Converter/LConn1
  gnd/RConn1 -- Voltage Sensor1/RConn2 -- Resistor2/RConn1 -- Capacitor1/RConn1 -- Voltage Sensor/RConn2 -- Resistor3/RConn1 -- Capacitor/RConn1
  Udc(-)/RConn1 -- Voltage Sensor1/LConn1 -- Capacitor1/LConn1 -- Resistor2/LConn1
  Udc(+)/RConn1 -- Voltage Sensor/LConn1 -- Resistor3/LConn1 -- Capacitor/LConn1

== system pgfm_ctrl_analysis/battery_1/single_phase_ui_measure ==
  Bus Creator : BusCreator  Inputs=2
  Current Sensor : fl_lib/Electrical/Electrical Sensors/Current Sensor
  Selector : Selector  InputPortWidth=2  IndexOptions=Index vector (dialog)  Indices=2  OutputSizes=1  RuntimeRangeChecks=off
  Selector1 : Selector  InputPortWidth=2  IndexOptions=Index vector (dialog)  Indices=1  OutputSizes=1  RuntimeRangeChecks=off
  Terminator : Terminator
  Terminator1 : Terminator
  Voltage Sensor : fl_lib/Electrical/Electrical Sensors/Voltage Sensor
  dab input modA : Scope  NumInputPorts=2
      settings: SampleTime=param.glb_time.tc  ActiveDisplayYMinimum=-469.43516743430069  ActiveDisplayYMaximum=519.37359595892747  DataLoggingVariableName=ScopeData2
  iph : nesl_utility/PS-Simulink Converter  PhysicalDomain=network_engine_domain  SubClassName=ps_output  LeftPortType=input  RightPortType=output  PseudoPeriodic=off  Frequencies=[]  VectorFormat=1-D array  Unit=A  AffineConversion=off
  uph : nesl_utility/PS-Simulink Converter  PhysicalDomain=network_engine_domain  SubClassName=ps_output  LeftPortType=input  RightPortType=output  PseudoPeriodic=off  Frequencies=[]  VectorFormat=1-D array  Unit=V  AffineConversion=off
  Udc(+) : PMIOPort  Side=Left
  udc(+) : PMIOPort  Port=2  Side=Right
  Udc(-) : PMIOPort  Port=3  Side=Left
  udc(-) : PMIOPort  Port=4  Side=Right
  tag scope: current_battery_1=global, voltage_battery_1=global
  wires:
  Bus Creator/1 -> Selector/1, Selector1/1  "ui_data"
  iph/1 -> Bus Creator/1  "iph"
  uph/1 -> Bus Creator/2  "uph"
  Selector1/1 -> [current_battery_1], dab input modA/1  "current_battery"
  Selector/1 -> dab input modA/2, [voltage_battery_1]  "voltage_battery"
  [current_battery_1] -> Terminator/1
  [voltage_battery_1] -> Terminator1/1
  connections:
  iph/LConn1 -- Current Sensor/RConn1
  Voltage Sensor/LConn1 -- Current Sensor/LConn1 -- Udc(+)/RConn1
  Current Sensor/RConn2 -- udc(+)/RConn1
  Voltage Sensor/RConn1 -- uph/LConn1
  Voltage Sensor/RConn2 -- Udc(-)/RConn1 -- udc(-)/RConn1

== system pgfm_ctrl_analysis/global timing/time_afe1 ==
  correction_time : Inport
  Constant : Constant
  Gain : Gain  Gain=k
  Product : Product
  Sum : Sum  Inputs=|++
  time_1 : Clock
  Out1 : Outport
  wires:
  time_1/1 -> Gain/1
  Gain/1 -> Product/1
  Product/1 -> Out1/1
  correction_time/1 -> Sum/1
  Sum/1 -> Product/2
  Constant/1 -> Sum/2

== system pgfm_ctrl_analysis/global timing/time_afe2 ==
  correction_time : Inport
  Constant : Constant
  Gain : Gain  Gain=k
  Product : Product
  Sum : Sum  Inputs=|++
  time_1 : Clock
  Out1 : Outport
  wires:
  time_1/1 -> Gain/1
  Gain/1 -> Product/1
  Product/1 -> Out1/1
  correction_time/1 -> Sum/1
  Constant/1 -> Sum/2
  Sum/1 -> Product/2

== system pgfm_ctrl_analysis/global timing/time_afe3 ==
  correction_time : Inport
  Constant : Constant
  Gain : Gain  Gain=k
  Product : Product
  Sum : Sum  Inputs=|++
  time_1 : Clock
  Out1 : Outport
  wires:
  Constant/1 -> Sum/2
  Sum/1 -> Product/2
  correction_time/1 -> Sum/1
  Product/1 -> Out1/1
  Gain/1 -> Product/1
  time_1/1 -> Gain/1

== system pgfm_ctrl_analysis/global timing/time_master ==
  Gain : Gain  Gain=k
  time_1 : Clock
  Out1 : Outport
  wires:
  Gain/1 -> Out1/1
  time_1/1 -> Gain/1

== system pgfm_ctrl_analysis/grid/grid_emulator ==
  3ph_Dyg_ssc : Subsystem
  Bus Selector : BusSelector  OutputSignals=ua_grid_emu,ub_grid_emu,uc_grid_emu
  Bus Selector1 : BusSelector  OutputSignals=gamma_grid_emulator,omega_grid_emulator
  Controlled Voltage Source : fl_lib/Electrical/Electrical Sources/Controlled Voltage Source
  Controlled Voltage Source1 : fl_lib/Electrical/Electrical Sources/Controlled Voltage Source
  Controlled Voltage Source2 : fl_lib/Electrical/Electrical Sources/Controlled Voltage Source
  Electrical Reference : fl_lib/Electrical/Electrical Elements/Electrical Reference
  Simulink-PS Converter : nesl_utility/Simulink-PS Converter  PhysicalDomain=network_engine_domain  SubClassName=ps_input  LeftPortType=input  RightPortType=output  PseudoPeriodic=off  Frequencies=[]  NoiseDistribution=none  NoiseParameters=[]  Unit=V  AffineConversion=on  FilteringAndDerivatives=provide  SimscapeFilterOrder=1  InputFilterTimeConstant=0.001  UdotUserProvided=0
  Simulink-PS Converter1 : nesl_utility/Simulink-PS Converter  PhysicalDomain=network_engine_domain  SubClassName=ps_input  LeftPortType=input  RightPortType=output  PseudoPeriodic=off  Frequencies=[]  NoiseDistribution=none  NoiseParameters=[]  Unit=V  AffineConversion=on  FilteringAndDerivatives=provide  SimscapeFilterOrder=1  InputFilterTimeConstant=0.001  UdotUserProvided=0
  Simulink-PS Converter2 : nesl_utility/Simulink-PS Converter  PhysicalDomain=network_engine_domain  SubClassName=ps_input  LeftPortType=input  RightPortType=output  PseudoPeriodic=off  Frequencies=[]  NoiseDistribution=none  NoiseParameters=[]  Unit=V  AffineConversion=on  FilteringAndDerivatives=provide  SimscapeFilterOrder=1  InputFilterTimeConstant=0.001  UdotUserProvided=0
  Solver Configuration : nesl_utility/Solver Configuration  PhysicalDomain=network_engine_domain  SubClassName=solver  LeftPortType=input  RightPortType=generic  Tones=[]  Harmonics=[]  SimulateNoise=off  Profile=off  UseLocalSampling=off  EnableSwitchedLinearOptims=on  FrequencyDomain=off  UseCCode=off  RelTol=0.001  AbsTol=0.001  MinStep=1e-09  ToWorkspace=off  RevertToSquareIcSolve=off  NumHomotopyIterations=100  PhasorMode=off  PhasorModeNumHarmonics=1  ConsistencySolver=NEWTON_FTOL  CanonicalOrdering=UNORDERED  OptimizeIntermediates=UNOPTIMIZED  MulticoreSolverChoice=BACKWARD_EULER  IndexReductionMethod=DerivativeReplacement  DoDC=off  ResidualTolerance=1e-4  ConsistencyTolSource=GLOBAL  ConsistencyAbsTol=0.001  ConsistencyRelTol=0.001  ConsistencyTolFactor=0.001  UseLocalSolver=on  LocalSolverChoice=NE_BACKWARD_EULER_ADVANCER  ResolveIndetEquations=on  FunctionEvalNumThread=1  LocalSolverSampleTime=param.glb_time.tc  DoFixedCost=on  MaxNonlinIter=param.sim.nonlinear_iterations  MaxModeIter=2  ComputeImpulses=off  ImpulseIterations=2  LinearAlgebra=auto  LinearAlgebraNumThread=0  EquationFormulation=NE_TIME_EF  DelaysMemoryBudget=1024  AutomaticFiltering=on  FilteringTimeConstant=0.001  PartitionStorageMethod=AS_NEEDED  PartitionMemoryBudget=1024  PartitionMethod=BALANCED  MultibodyUseLocalSolver=off  MultibodyLocalSolverChoice=ODE1  MultibodyLocalSolverSampleTime=0.001
  td2tc_1 : TransferFcn  Denominator=[param.glb_time.tc 1]
  td2tc_2 : TransferFcn  Denominator=[param.glb_time.tc 1]
  td2tc_3 : TransferFcn  Denominator=[param.glb_time.tc 1]
  three_phase_voltage_source_with_frt_emulator1 : three_phase_voltage_with_frt_emulator_mfcn/three_phase_voltage_source_with_frt_emulator  nominal_frequency_m=param.grid.emu.fgrid_nom  nominal_voltage_m=param.grid.emu.us_secondary_nom  Vemu_ref_norm_m=param.grid.emu.Vemu_ref_norm  vp_xi_pu_m=param.grid.emu.up_xi_pu_ref  vp_eta_pu_m=param.grid.emu.up_eta_pu_ref  vn_xi_pu_m=param.grid.emu.un_xi_pu_ref  vn_eta_pu_m=param.grid.emu.un_eta_pu_ref  Am=param.ctrl.filters.afe.SOF_50Hz.ss_c.A  Bm=param.ctrl.filters.afe.SOF_50Hz.ss_c.B  Cm=param.ctrl.filters.afe.SOF_50Hz.ss_c.C  enable_frt_1_m=param.frt.data.enable_frt_1  enable_frt_2_m=param.frt.data.enable_frt_2  start_time_LVRT_m=param.frt.data.start_time_LVRT  end_time_LVRT_m=param.frt.data.end_time_LVRT  deepPOSxi_m=param.frt.data.deepPOSxi  deepPOSeta_m=param.frt.data.deepPOSeta  deepNEGxi_m=param.frt.data.deepNEGxi  deepNEGeta_m=param.frt.data.deepNEGeta  Amplitude_U_m=param.frt.data.Amplitude_U  Amplitude_V_m=param.frt.data.Amplitude_V  Amplitude_W_m=param.frt.data.Amplitude_W  t_ramp_m=param.frt.data.t_ramp  Phase_shift_m=param.frt.data.Phase_shift
  threephase_vi_measures : Subsystem
  u1 : PMIOPort  Side=Right
  u2 : PMIOPort  Port=2  Side=Right
  u3 : PMIOPort  Port=3  Side=Right
  tag scope: omega_grid_emulator=global, phase_grid_emulator=global
  wires:
  Bus Selector1/2 -> [omega_grid_emulator]  "<omega_grid_emulator>"
  Bus Selector1/1 -> [phase_grid_emulator]  "<gamma_grid_emulator>"
  Bus Selector/2 -> td2tc_2/1  "<ub_grid_emu>"
  Bus Selector/3 -> td2tc_3/1  "<uc_grid_emu>"
  three_phase_voltage_source_with_frt_emulator1/1 -> Bus Selector1/1, Bus Selector/1
  Bus Selector/1 -> td2tc_1/1  "<ua_grid_emu>"
  td2tc_1/1 -> Simulink-PS Converter/1  "ua(t)"
  td2tc_2/1 -> Simulink-PS Converter1/1  "ub(t)"
  td2tc_3/1 -> Simulink-PS Converter2/1  "uc(t)"
  connections:
  Simulink-PS Converter/RConn1 -- Controlled Voltage Source/RConn1
  Simulink-PS Converter1/RConn1 -- Controlled Voltage Source1/RConn1
  Simulink-PS Converter2/RConn1 -- Controlled Voltage Source2/RConn1
  Electrical Reference/LConn1 -- Controlled Voltage Source/RConn2 -- Controlled Voltage Source1/RConn2 -- Controlled Voltage Source2/RConn2 -- Solver Configuration/RConn1
  3ph_Dyg_ssc/RConn1 -- u1/RConn1
  3ph_Dyg_ssc/RConn2 -- u2/RConn1
  3ph_Dyg_ssc/RConn3 -- u3/RConn1
  3ph_Dyg_ssc/LConn1 -- threephase_vi_measures/RConn1
  3ph_Dyg_ssc/LConn2 -- threephase_vi_measures/RConn2
  3ph_Dyg_ssc/LConn3 -- threephase_vi_measures/RConn3
  Controlled Voltage Source/LConn1 -- threephase_vi_measures/LConn1
  Controlled Voltage Source1/LConn1 -- threephase_vi_measures/LConn2
  Controlled Voltage Source2/LConn1 -- threephase_vi_measures/LConn3
